simulink subsystem "VehSpdRef_Basic_refsub"  (R2025a)
settings: Solver=VariableStepAuto  StartTime=0.0  StopTime=10.0  RelTol=1e-3
libraries: simulink x3, autolibshared x1
settings Model: Creator=isaacito  LastModifiedBy=isaacito
settings OptimizationCC: ReuseModelBlockBuffer=off
settings RTWCC: GPUComputeCapability=3.5

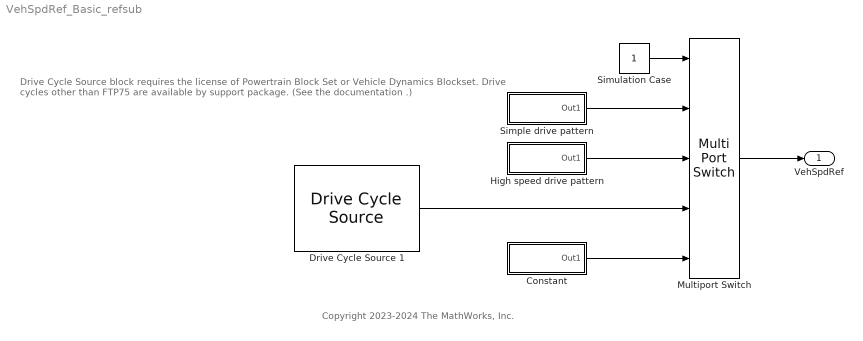
== system VehSpdRef_Basic_refsub ==
  note: Drive Cycle Source block requires the license of Powertrain Block Set
      | or Vehicle Dynamics Blockset.
      | Drive cycles other than FTP75 are available by support package.
      | (See the documentation .)
  note: Copyright 2023-2024 The MathWorks, Inc.
  Constant : Subsystem  mask(Continuous Multi-Step Signal){dataPoints=[0 1000 0], deltaT=0.5}
      mask prompts: dataPoints "Data points"; deltaT "Interpolation step [s]"
      mask help:
      | This block generates a signal consisting of smoothly connected flat segments. Data points parameter takes an N-by-3 matrix where each row specifies a flat segment. First column and second column define start and end time of the segment, respectively. Third column defines the value of the segment. Second column can also be NaN to define a point value. Flat segments and point values are smoothly interpolated by Akima spline with the specified interpolation step.
      |
      | For example, a matrix [0 1 5; 3 nan 9; 6 8 7] for Data points defines a signal as follows. First row defines a flat segment from t=0 to t=1 of value 5. Second row defines a point at t=3 of value 9. Third row defines a flat segment from t=6 to t=8 of value 7.
      mask init:
      | sig = SignalDesigner("ContinuousMultiStep");
      | 
      | % Initialization function can access parameter names directly
      | sig.XYData = dataPoints;
      | sig.DeltaX = deltaT;
      | 
      | update(sig)
      mask DialogControl Control3 Prompt: horizontal spacer 1
      mask DialogControl Control4 Prompt: horizontal spacer 2
      mask DialogControl Control5 Prompt: horizontal spacer 3
      mask DialogControl PlotButton Prompt: Plot
      mask DialogControl PlotButton Callback: SignalSourceBlockCallback.plotContinuousMultiStep(gcb);
      mask Display: disp("Continuous" + newline + "Multi-Step")
  Drive Cycle Source 1 : autolibshared/Drive Cycle Source  cycleVar=FTP75  fileVar=cycleFTP75.mat  tfinal="2474  seconds"  cycleRepeat=off  outAccPort=off  outGearPort=off  gearList=No gear data  t_wot1=5  xdot_woto=0  xdot_wot1=30  t_wot2=20  xdot_wot2=0  t_wotend=30  srcUnit=m/s  outUnit=km/h  srcAccUnit=m/s/s  outAccUnit=m/s^2  dt=0  aMode=1  faultOption=off  velBnd=2  velBndUnit=mph  inUnit=m/s  timeBnd=1  failOption=off  stopSim=off  maxFaultCnt=10  maxFaultTime=2  maxTotFaultTime=15  traceOption=off  dtTrace=1  traceWindow=10  lastDCname=FTP75  lastOutUnit=mph  lastDT=0  lastTB=1  lastSB=2  forceCalcBound=off
  High speed drive pattern : Subsystem  mask(Trace Generator){yScale=1, tScale=1, randomSeed=6, interpolationStepSize=0.5, tInitialFlatLength=10, yInitialValue=0, numTransitions=10, transitionRange=[5 10], flatRange=[5 10], yRange=[60 100], tFinalTransitionDuration=15, tFinalFlatDuration=10, yFinalValue=0}
      mask prompts: yScale "Data value scaler"; tScale "Time scaler"; randomSeed "Random seed"; interpolationStepSize "Interpolation step [s]"; tInitialFlatLength "Initial constant duration"; yInitialValue "Initial data value"; numTransitions "Number of transitions"; transitionRange "Range of transition duration"; flatRange "Range of constant duration"; yRange "Range of data value"; tFinalTransitionDuration "Final transition duration"; tFinalFlatDuration "Final constant duration"; yFinalValue "Final data value"
      mask help: This block generates a smooth signal consisting of flat segments.
      mask init:
      | xydata = SignalDesignUtility.buildXYData( ...
      |   RandomSeed = randomSeed, ...
      |   XScale = tScale, ...
      |   YScale = yScale, ...
      |   XInitialFlatLength = tInitialFlatLength, ...
      |   YInitialValue = yInitialValue, ...
      |   NumTransitions  = numTransitions, ...
      |   TransitionRange = transitionRange, ...
      |   FlatRange = flatRange, ...
      |   YRange = yRange, ...
      |   XFinalTransitionLength = tFinalTransitionDuration, ...
      |   XFinalFlatLength = tFinalFlatDuration, ...
      |   YFinalValue = yFinalValue );
      | 
      | sig = SignalDesigner("ContinuousMultiStep");
      | sig.XYData = xydata;
      | sig.DeltaX = interpolationStepSize;
      | 
      | update(sig)
      mask DialogControl Container3 Prompt: Advanced
      mask DialogControl Control3 Prompt: horizontal spacer 1
      mask DialogControl Control4 Prompt: horizontal spacer 2
      mask DialogControl Control5 Prompt: horizontal spacer 3
      mask DialogControl PlotButton Prompt: Plot
      mask DialogControl PlotButton Callback: SignalSourceBlockCallback.plotTraceGenerator(gcb);
      mask Display: disp("Trace" + newline + "Generator")
  Multiport Switch : MultiPortSwitch  Inputs=4  SaturateOnIntegerOverflow=off  InputSameDT=off
  Simple drive pattern : Subsystem  mask(Continuous Multi-Step Signal){dataPoints=[0 10 0; 15 25 20; 30 nan 45; 45 50 70; 70 nan 50; 95 100 0], deltaT=0.5}
      mask prompts: dataPoints "Data points"; deltaT "Interpolation step [s]"
      mask help:
      | This block generates a signal consisting of smoothly connected flat segments. Data points parameter takes an N-by-3 matrix where each row specifies a flat segment. First column and second column define start and end time of the segment, respectively. Third column defines the value of the segment. Second column can also be NaN to define a point value. Flat segments and point values are smoothly interpolated by Akima spline with the specified interpolation step.
      |
      | For example, a matrix [0 1 5; 3 nan 9; 6 8 7] for Data points defines a signal as follows. First row defines a flat segment from t=0 to t=1 of value 5. Second row defines a point at t=3 of value 9. Third row defines a flat segment from t=6 to t=8 of value 7.
      mask init:
      | sig = SignalDesigner("ContinuousMultiStep");
      | 
      | % Initialization function can access parameter names directly
      | sig.XYData = dataPoints;
      | sig.DeltaX = deltaT;
      | 
      | update(sig)
      mask DialogControl Control3 Prompt: horizontal spacer 1
      mask DialogControl Control4 Prompt: horizontal spacer 2
      mask DialogControl Control5 Prompt: horizontal spacer 3
      mask DialogControl PlotButton Prompt: Plot
      mask DialogControl PlotButton Callback: SignalSourceBlockCallback.plotContinuousMultiStep(gcb);
      mask Display: disp("Continuous" + newline + "Multi-Step")
  Simulation Case : Constant
  VehSpdRef : Outport  Unit=km/h
      settings: AttributesFormatString=%<Unit>
  wires:
  Drive Cycle Source 1/1 -> Multiport Switch/4
  High speed drive pattern/1(Out1) -> Multiport Switch/3
  Simple drive pattern/1(Out1) -> Multiport Switch/2
  Simulation Case/1 -> Multiport Switch/1
  Multiport Switch/1 -> VehSpdRef/1
  Constant/1(Out1) -> Multiport Switch/5

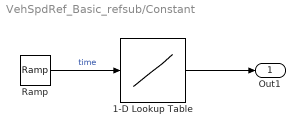
== system VehSpdRef_Basic_refsub/Constant ==
  1-D Lookup Table : Lookup_n-D  NumberOfTableDimensions=1  BreakpointsForDimension1=sig.Data.X  Table=sig.Data.Y  InternalRulePriority=Speed  RndMeth=Simplest
  Ramp : simulink/Sources/Ramp  slope=1  start=0  InitialOutput=0
      settings: AttributesFormatString=|
      | Slope: %<slope>
      | Start time: %<start>
      | Initial output: %<InitialOutput>
  Out1 : Outport
  wires:
  Ramp/1 -> 1-D Lookup Table/1  "time"
  1-D Lookup Table/1 -> Out1/1

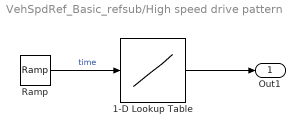
== system VehSpdRef_Basic_refsub/High speed drive pattern ==
  1-D Lookup Table : Lookup_n-D  NumberOfTableDimensions=1  BreakpointsForDimension1=sig.Data.X  Table=sig.Data.Y  InternalRulePriority=Speed  RndMeth=Simplest
  Ramp : simulink/Sources/Ramp  slope=1  start=0  InitialOutput=0
      settings: AttributesFormatString=|
      | Slope: %<slope>
      | Start time: %<start>
      | Initial output: %<InitialOutput>
  Out1 : Outport
  wires:
  1-D Lookup Table/1 -> Out1/1
  Ramp/1 -> 1-D Lookup Table/1  "time"

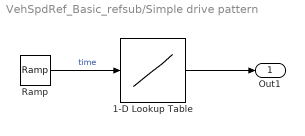
== system VehSpdRef_Basic_refsub/Simple drive pattern ==
  1-D Lookup Table : Lookup_n-D  NumberOfTableDimensions=1  BreakpointsForDimension1=sig.Data.X  Table=sig.Data.Y  InternalRulePriority=Speed  RndMeth=Simplest
  Ramp : simulink/Sources/Ramp  slope=1  start=0  InitialOutput=0
      settings: AttributesFormatString=|
      | Slope: %<slope>
      | Start time: %<start>
      | Initial output: %<InitialOutput>
  Out1 : Outport
  wires:
  Ramp/1 -> 1-D Lookup Table/1  "time"
  1-D Lookup Table/1 -> Out1/1
